simulink model "global_In"  (R2025b)
settings: Solver=VariableStepAuto  StartTime=0.0  StopTime=10.0  RelTol=1e-3
settings Model: Creator=EMK7KOR  LastModifiedBy=EMK7KOR

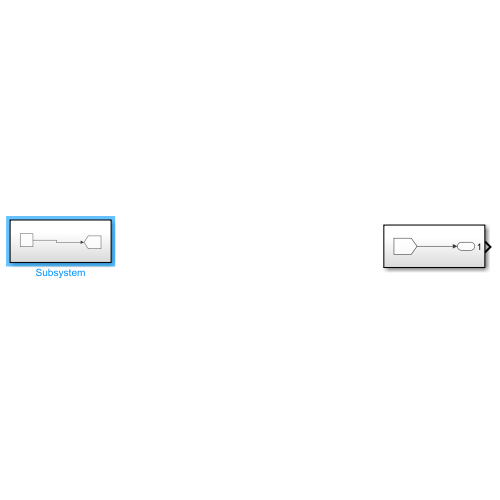
[thumbnail: Simulink's stored preview of the top-level diagram]
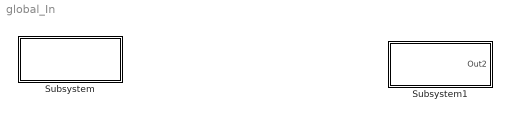
== system global_In ==
  Subsystem : Subsystem
  Subsystem1 : Subsystem

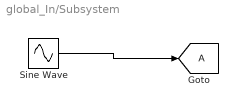
== system global_In/Subsystem ==
  Goto : Goto  TagVisibility=global
  Sine Wave : Sin  SampleTime=0
  wires:
  Sine Wave/1 -> Goto/1

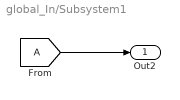
== system global_In/Subsystem1 ==
  From : From  TagVisibility=global
  Out2 : Outport
  wires:
  From/1 -> Out2/1
